simulink model "sschdlexZVSResonantConverterModel"  (R2026a)
settings: Solver=FixedStepDiscrete  StopTime=0.0001
libraries: fl_lib x9, nesl_utility x8, ee_lib x2
settings Model: DataTypeOverride=Off  Creator=The MathWorks, Inc.  LastModifiedBy=The MathWorks, Inc.
settings OptimizationCC: ConditionallyExecuteInputs=off
settings DebuggingCC: AlgebraicLoopMsg=error  SingleTaskRateTransMsg=error
settings HardwareCC: ProdHWDeviceType=ASIC/FPGA->ASIC/FPGA  TargetBitPerLong=64.0  TargetBitPerPointer=64.0  TargetBitPerSizeT=64.0  TargetBitPerPtrDiffT=64.0  TargetLongLongMode=on  TargetIntDivRoundTo=Zero  TargetEndianess=LittleEndian  TargetWordSize=64.0  TargetHWDeviceType=Custom Processor->MATLAB Host Computer  ProdEqTarget=off
settings SimscapeCC: SimscapeNominalValues="[{\"value\":\"1\",\"unit\":\"A\"},{\"value\":\"1\",\"unit\":\"bar\"},{\"value\":\"1\",\"unit\":\"cm^2\"},{\"value\":\"1\",\"unit\":\"cm^3/s\"},{\"value\":\"1\",\"unit\":\"kJ/kg\"},{\"value\":\"1\",\"unit\":\"kW\"},{\"value\":\"1\",\"unit\":\"l\"},{\"value\":\"1\",\"unit\":\"N\"},{\"value\":\"1\",\"unit\":\"N*m\"},{\"value\":\"1\",\"unit\":\"V\"}]"  SimscapeLogType=none  SimscapeLogDataHistory=5000.0

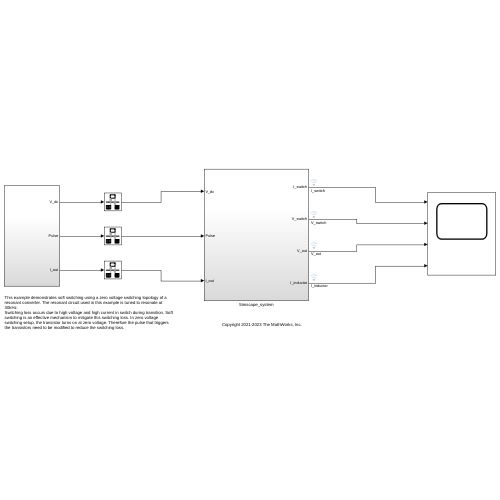
[thumbnail: Simulink's stored preview of the top-level diagram]
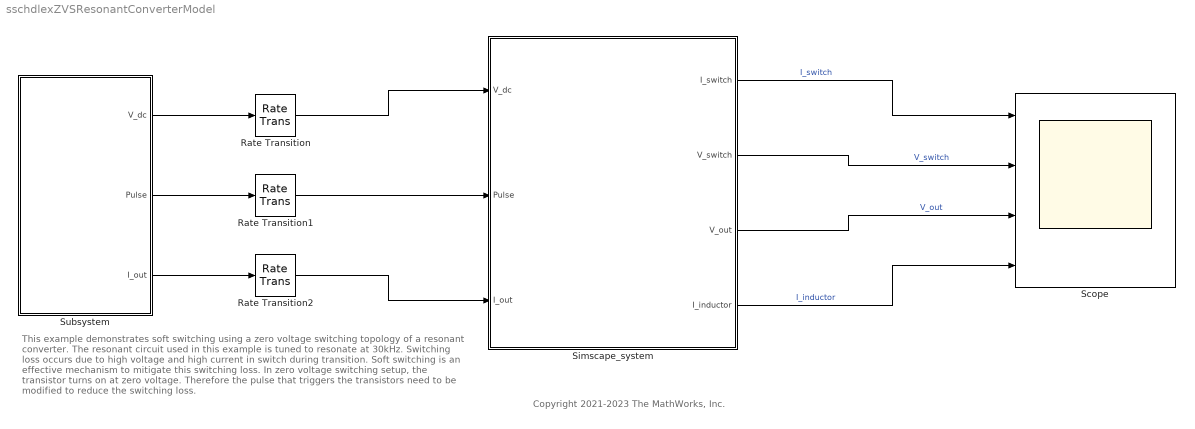
== system sschdlexZVSResonantConverterModel ==
  note: This example demonstrates soft switching using a zero voltage switching topology of a resonant converter. The resonant circuit used in this example is tuned to resonate at 30kHz.
      | Switching loss occurs due to high voltage and high current in switch during transition. Soft switching is an effective mechanism to mitigate this switching loss. In zero voltage switching setup, the transistor turns on at zero voltage. Therefore the pulse that triggers the transistors need to be modified to reduce the switching loss.
  note: Copyright 2021-2023 The MathWorks, Inc.
  Rate Transition : RateTransition
  Rate Transition1 : RateTransition
  Rate Transition2 : RateTransition
  Scope : Scope  NumInputPorts=4
      settings: ActiveDisplayYMinimum=-0.125  ActiveDisplayYMaximum=1.125
  Simscape_system : Subsystem
  Subsystem : Subsystem
  wires:
  Subsystem/1(V_dc) -> Rate Transition/1
  Subsystem/2(Pulse) -> Rate Transition1/1
  Subsystem/3(I_out) -> Rate Transition2/1
  Rate Transition/1 -> Simscape_system/1(V_dc)
  Rate Transition1/1 -> Simscape_system/2(Pulse)
  Rate Transition2/1 -> Simscape_system/3(I_out)
  Simscape_system/1(I_switch) -> Scope/1  "I_switch"
  Simscape_system/2(V_switch) -> Scope/2  "V_switch"
  Simscape_system/3(V_out) -> Scope/3  "V_out"
  Simscape_system/4(I_inductor) -> Scope/4  "I_inductor"

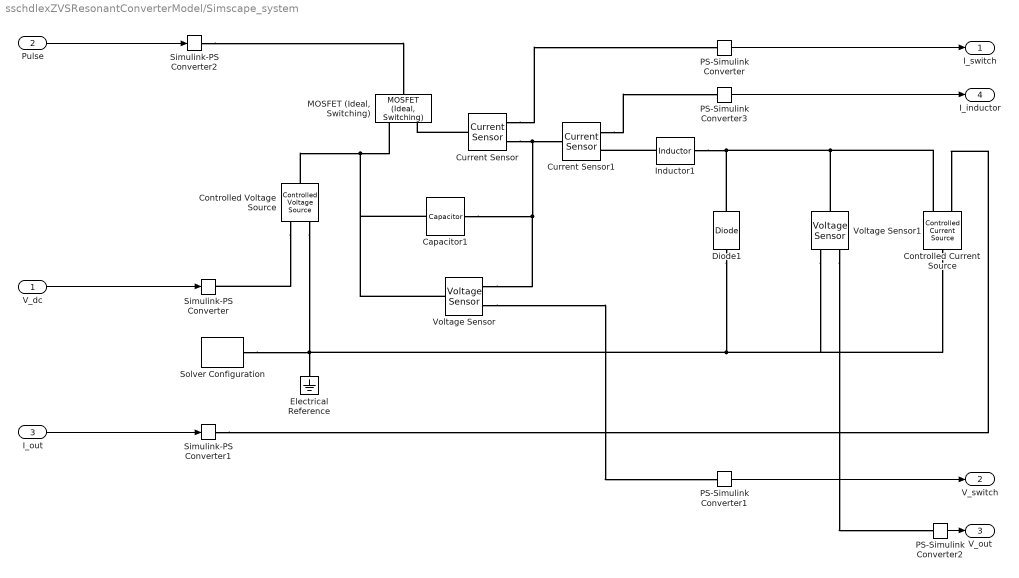
== system sschdlexZVSResonantConverterModel/Simscape_system ==
  V_dc : Inport
  Pulse : Inport  Port=2
  I_out : Inport  Port=3
  Capacitor1 : fl_lib/Electrical/Electrical Elements/Capacitor  c=0.1e-6 F  r=1e-6 Ohm  g=0 1/Ohm  i_specify=off  i_priority=None  i=0 A  i_nominal_specify=off  i_nominal_value=1  i_nominal_unit=A  v_specify=off  v_priority=None  v=0 V  v_nominal_specify=off  v_nominal_value=1  v_nominal_unit=V  vc_specify=off  vc_priority=High  vc=0 V  vc_nominal_specify=off  vc_nominal_value=1  vc_nominal_unit=V
  Controlled Current Source : fl_lib/Electrical/Electrical Sources/Controlled Current Source
  Controlled Voltage Source : fl_lib/Electrical/Electrical Sources/Controlled Voltage Source
  Current Sensor : fl_lib/Electrical/Electrical Sensors/Current Sensor
  Current Sensor1 : fl_lib/Electrical/Electrical Sensors/Current Sensor
  Diode1 : ee_lib/Semiconductors & Converters/Diode  ModelType=ee.enum.diode.modelType.pwl  TableType=ee.enum.diode.tableType.IfMat  IfMat=[.07, .12, .19, 1.75, 4.24, 7.32, 11.2; .16, .3, .72, 2.14, 5.02, 8.35, 13.12] A  VfMat=[.9, 1.15, 1.25, 1.5, 1.75, 2.17, 2.6, 2.85; .58, .68, .75, 1.1, 1.38, 1.77, 2.27, 2.7] V  TjVec=[25, 125] degC  VfVec=[.5, .7, .9, 1.3, 1.7, 2.1, 2.5] V  IfVec=[.1, .2, .5, 1, 2, 4, 7, 10] A  IrMat=[1e-06, 2e-06, 5e-06, 1e-05, 2.5e-05, 5e-05, .0001; 2e-06, 5e-06, 1e-05, 4e-05, 8e-05, .0002, .0005] A  VrMat=[10, 100, 200, 250, 300, 325, 350; 10, 70, 160, 220, 270, 300, 320] V  VrVec=[10, 20, 40, 50, 70, 80, 100] V  IrVec=[1e-06, 2e-06, 5e-06, 1e-05, 2e-05, 5e-05, .0001] A  Vf=0.6 V  Ron=0.3 Ohm  Goff=1e-8 S  prmExp=ee.enum.diode.expParam.useTwo  I12=[.0137, .545] A  V12=[.6, .7] V  RS=0 Ohm  Tmeas=25 degC  IS=1e-12 A  ec=1  I1=0.0137 A  V1=0.6 V  N_series=1  N_parallel=1  ZenerEnable=false  Rz=0.3 Ohm  BV=inf V  C_param=ee.enum.diode.capParam.fixed  CJ=0 pF  CJ0=5 pF  Vvec=[.1, 10, 100] V  Cvec=[3.5, 1, .4] pF  VJ=1 V  Mgrad=0.5  FC=0.5  Q_param=ee.enum.diode.recoveryParam.off  iRM=-7.15 A  iF=4 A  didt=-750 A/us  trr_factor=3  trr=115 ns  Qrr=150 nA*s  Vr=-600 V  Ls=150 nH  Erec=0.03 J  TT=50 ns  tau=100 ns  T_param=ee.enum.diode.temperatureParam.off  Tdevice=25 degC  I1_T2=0.245 A  V1_T2=0.5 V  IS_T2=1.25e-7 A  Tmeas2=125 degC  XTI_param=ee.enum.diode.xtiParam.pn  XTI=3  EG_param=ee.enum.diode.egapParam.material_si  EG=1.11 eV  dBVdT=0 V/K  enable_fault_input=simscape.enum.onoff.off  i_specify=off  i_priority=None  i=0 A  i_nominal_specify=off  i_nominal_value=1  i_nominal_unit=A  v_specify=off  v_priority=None  v=0 V  v_nominal_specify=off  v_nominal_value=1  v_nominal_unit=V  v_capacitor_specify=off  v_capacitor_priority=None  v_capacitor=0 V  v_capacitor_nominal_specify=off  v_capacitor_nominal_value=1  v_capacitor_nominal_unit=V  Qj_specify=off  Qj_priority=High  Qj=0 C  Qj_nominal_specify=off  Qj_nominal_value=1  Qj_nominal_unit=C  i_diode_specify=off  i_diode_priority=None  i_diode=0 A  i_diode_nominal_specify=off  i_diode_nominal_value=1  i_diode_nominal_unit=A  v_diode_specify=off  v_diode_priority=None  v_diode=0 V  v_diode_nominal_specify=off  v_diode_nominal_value=1  v_diode_nominal_unit=V  i_capacitor_specify=off  i_capacitor_priority=None  i_capacitor=0 A  i_capacitor_nominal_specify=off  i_capacitor_nominal_value=1  i_capacitor_nominal_unit=A  fidelity_level=ee.enum.diode.fidelity.includeChargeDyn  rec_loss_model=ee.enum.diode.reverseRecoveryModel.fixed  ErecVal=0 J  scaleWithIandV=true  ErecMat=zeros(2, 3) J  ErecMat3D=zeros(2, 3, 2) J  TjrecVec=[298.15, 398.15] K  IfrecVec=[.1, 1, 10] A  IrecVal=10 A  VrecVal=10 V  VrecVec=[0, 100] V  tFilter=1 / 1000 / 100 s  thermal_network_parameterization=ee.enum.thermalNetworkTopology.junctionCase  Rth=[0, 10] K/W  Rth_Cauer=[1, 3, 10] K/W  Rth_Foster=[4, 6] K/W  thermal_mass_parameterization=ee.enum.thermalNetwork.timeconstant  thermal_mass=[0, 1] J/K  thermal_mass_Cauer=[.1, .3, 1] J/K  thermal_mass_Foster=[1.5, 3] J/K  thermal_time_constant=[0, 10] s  thermal_time_constant_Cauer=[1, 3, 10] s  thermal_time_constant_Foster=[6, 18] s  thermal_mass_initial_temperatures=[25, 25] degC  thermal_mass_initial_temperatures_Cauer=[25, 25, 25] degC  junction_thermal_mass=0.01 J/K  Tvec_initial_Foster=[25, 25, 25, 25] degC  no_thermal_network=0  junction_temperature_specify=off  junction_temperature_priority=None  junction_temperature=25 degC  junction_temperature_nominal_specify=off  junction_temperature_nominal_value=1  junction_temperature_nominal_unit=degC
  Electrical Reference : fl_lib/Electrical/Electrical Elements/Electrical Reference
  Inductor1 : fl_lib/Electrical/Electrical Elements/Inductor  l=0.1e-3 H  r=0 Ohm  g=1e-9 1/Ohm  i_specify=on  i_priority=None  i=1 A  i_nominal_specify=off  i_nominal_value=1  i_nominal_unit=A  v_specify=off  v_priority=None  v=0 V  v_nominal_specify=off  v_nominal_value=1  v_nominal_unit=V  i_L_specify=off  i_L_priority=High  i_L=0 A  i_L_nominal_specify=off  i_L_nominal_value=1  i_L_nominal_unit=A
  "MOSFET (Ideal, Switching)" : ee_lib/Semiconductors & Converters/MOSFET (Ideal, Switching)  port_option=ee.enum.controlport.ps  Rds=1 Ohm  Goff=1e-6 1/Ohm  Vth=0.7 V  diode_param=2  diode_Vf=0.8 V  diode_Ron=0.001 Ohm  diode_Goff=1e-5 1/Ohm  diode_C=50e-9 F  diode_iRM=-235 A  diode_iF=300 A  diode_idot=-50 A/us  diode_trr_param=1  diode_trr_factor=3  diode_trr=15 us  diode_Qrr=1500 s*uA  ids_specify=off  ids_priority=None  ids=0 A  ids_nominal_specify=off  ids_nominal_value=1  ids_nominal_unit=A  vds_specify=off  vds_priority=None  vds=0 V  vds_nominal_specify=off  vds_nominal_value=1  vds_nominal_unit=V  vgs_specify=off  vgs_priority=None  vgs=0 V  vgs_nominal_specify=off  vgs_nominal_value=1  vgs_nominal_unit=V  thermal_loss_option=ee.enum.converters.thermalLossOption.constantvalues  Von_data=[0, 1.8, 3.2, 6, 10, 16; 0, 2, 5.5, 9.5, 15, 25] V  Tj=[298.15, 448.15] K  Iout_data=[0, 20, 40, 60, 80, 100] A  tabulateWithVds=false  Eon_data=[0, 55.04, 124.57, 235.53, 362.12; 0, 71.25, 161.25, 304.88, 468.75] * 1e-6 J  Eoff_data=[0, 18, 30, 56.1, 76.5; 0, 22.5, 37.5, 70.13, 95.63] * 1e-6 J  Eon_data_3D=[zeros(2, 5, 3)] J  Eoff_data_3D=[zeros(2, 5, 3)] J  Tj_loss=[298.15, 448.15] K  Iout_data_loss=[0, 10, 20, 30, 40] A  Vds_loss=[0, 150, 300] V  Eon_scalar=22.86e-3 J  Eoff_scalar=17.14e-3 J  Voff=300 V  Iout_scalar=600 A  useCurrentFromPreviousCycle=false  useVoltageFromPreviousCycle=false  diodeModelType=ee.enum.converters.diodeModelType.pwl  diodeTableType=ee.enum.diode.tableType.IfMat  diode_ReverseIVType=ee.enum.diode.diodeReverseIV.constant  diode_IfMat=[.07, .12, .19, 1.75, 4.24, 7.32, 11.2; .16, .3, .72, 2.14, 4.02, 6.35, 9.12] A  diode_VfMat=[.9, 1.15, 1.25, 1.5, 1.75, 2.17, 2.6, 2.85; .58, .68, .75, 1.1, 1.38, 1.77, 2.27, 2.7] V  diode_TjVec=[25, 125] degC  diode_VfVec=[.5, .7, .9, 1.3, 1.7, 2.1, 2.5] V  diode_IfVec=[.1, .2, .5, 1, 2, 4, 7, 10] A  diode_IrMat=[1e-06, 2e-06, 5e-06, 1e-05, 2.5e-05, 5e-05, .0001; 2e-06, 5e-06, 1e-05, 4e-05, 8e-05, .0002, .0005] A  diode_VrMat=[10, 100, 200, 250, 300, 325, 350; 10, 70, 160, 220, 270, 300, 320] V  diode_VrVec=[10, 20, 40, 50, 70, 80, 100] V  diode_IrVec=[1e-06, 2e-06, 5e-06, 1e-05, 2e-05, 5e-05, .0001] A  diode_Vr=-600 V  diode_Ls=150 nH  diode_Erec=0.03 J  diode_rec_loss_model=ee.enum.diode.reverseRecoveryModel.fixed  diode_ErecVal=0 J  diode_scaleWithIandV=true  diode_ErecMat=zeros(2, 3) J  diodeErecMat3D=zeros(2, 3, 2) J  diode_TjrecVec=[298.15, 398.15] K  diode_IfrecVec=[.1, 1, 10] A  diodeVrecVec=[0, 100] V  diode_IrecVal=10 A  diode_VrecVal=10 V  diode_tFilter=1 / 1000 / 100 s  separateThermalPortForDiode=false  thermal_network_parameterization=ee.enum.thermalNetworkTopology.external  Rth=[.03, .2] K/W  Rth_Cauer=[.03, .1, .2] K/W  Rth_Foster=[.03, .2] K/W  thermal_mass_parameterization=ee.enum.thermalNetwork.timeconstant  thermal_mass=[3, 25] J/K  thermal_mass_Cauer=[3, 10, 25] J/K  thermal_mass_Foster=[33, 50] J/K  thermal_time_constant=[.1, 5] s  thermal_time_constant_Cauer=[.1, 1, 5] s  thermal_time_constant_Foster=[1, 10] s  thermal_mass_initial_temperatures=[25, 25] degC  thermal_mass_initial_temperatures_Cauer=[25, 25, 25] degC  junction_thermal_mass=0.1 J/K  Tvec_initial_Foster=[25, 25, 25, 25] degC  RthDiode=[.03, .2] K/W  RthCauerDiode=[.03, .1, .2] K/W  RthFosterDiode=[.03, .2] K/W  thermalMassDiode=[3, 25] J/K  thermalMassCauerDiode=[3, 10, 25] J/K  thermalMassFosterDiode=[33, 50] J/K  thermalTauDiode=[.1, 5] s  thermalTauCauerDiode=[.1, 1, 5] s  thermalTauFosterDiode=[1, 10] s  thermalMassInitTempDiode=[25, 25] degC  thermalMassInitTempCauerDiode=[25, 25, 25] degC  junctionthermalMassDiode=0.1 J/K  TVecInitialFosterDiode=[25, 25, 25, 25] degC  no_thermal_network=0  mosfet_junction_temperature_specify=off  mosfet_junction_temperature_priority=None  mosfet_junction_temperature=25 degC  mosfet_junction_temperature_nominal_specify=off  mosfet_junction_temperature_nominal_value=1  mosfet_junction_temperature_nominal_unit=degC  diode_junction_temperature_specify=off  diode_junction_temperature_priority=None  diode_junction_temperature=25 degC  diode_junction_temperature_nominal_specify=off  diode_junction_temperature_nominal_value=1  diode_junction_temperature_nominal_unit=degC  Qj_specify=off  Qj_priority=None  Qj=0 W  Qj_nominal_specify=off  Qj_nominal_value=1  Qj_nominal_unit=W  accumulatedSwitchingLosses_specify=off  accumulatedSwitchingLosses_priority=None  accumulatedSwitchingLosses=0 J
  PS-Simulink Converter{,1..3} (4 alike) : nesl_utility/PS-Simulink Converter  PhysicalDomain=network_engine_domain  SubClassName=ps_output  LeftPortType=input  RightPortType=output  PseudoPeriodic=off  Frequencies=[]  VectorFormat=1-D array  Unit=inherit  AffineConversion=off
  Simulink-PS Converter : nesl_utility/Simulink-PS Converter  PhysicalDomain=network_engine_domain  SubClassName=ps_input  LeftPortType=input  RightPortType=output  PseudoPeriodic=off  Frequencies=[]  NoiseDistribution=none  NoiseParameters=[]  Unit=1  AffineConversion=off  FilteringAndDerivatives=provide  SimscapeFilterOrder=1  InputFilterTimeConstant=0.001  UdotUserProvided=0
  Simulink-PS Converter1 : nesl_utility/Simulink-PS Converter  PhysicalDomain=network_engine_domain  SubClassName=ps_input  LeftPortType=input  RightPortType=output  PseudoPeriodic=off  Frequencies=[]  NoiseDistribution=none  NoiseParameters=[]  Unit=1  AffineConversion=off  FilteringAndDerivatives=provide  SimscapeFilterOrder=1  InputFilterTimeConstant=0.001  UdotUserProvided=0
  Simulink-PS Converter2 : nesl_utility/Simulink-PS Converter  PhysicalDomain=network_engine_domain  SubClassName=ps_input  LeftPortType=input  RightPortType=output  PseudoPeriodic=off  Frequencies=[]  NoiseDistribution=none  NoiseParameters=[]  Unit=1  AffineConversion=off  FilteringAndDerivatives=provide  SimscapeFilterOrder=1  InputFilterTimeConstant=0.001  UdotUserProvided=0
  Solver Configuration : nesl_utility/Solver Configuration  PhysicalDomain=network_engine_domain  SubClassName=solver  LeftPortType=input  RightPortType=generic  Tones=[]  Harmonics=[]  SimulateNoise=off  Profile=off  UseLocalSampling=off  EnableSwitchedLinearOptims=on  FrequencyDomain=off  UseCCode=off  RelTol=0.001  AbsTol=1e-06  MinStep=1e-09  ToWorkspace=off  RevertToSquareIcSolve=off  NumHomotopyIterations=100  PhasorMode=off  PhasorModeNumHarmonics=1  ConsistencySolver=NEWTON_FTOL  CanonicalOrdering=UNORDERED  OptimizeIntermediates=UNOPTIMIZED  IndexReductionMethod=DerivativeReplacement  DoDC=off  ResidualTolerance=1e-09  ConsistencyTolSource=GLOBAL  ConsistencyAbsTol=0.001  ConsistencyRelTol=0.001  ConsistencyTolFactor=0.001  UseLocalSolver=on  LocalSolverChoice=NE_BACKWARD_EULER_ADVANCER  ResolveIndetEquations=on  FunctionEvalNumThread=1  LocalSolverSampleTime=1e-6  DoFixedCost=on  MaxNonlinIter=2  MaxModeIter=2  ComputeImpulses=off  ImpulseIterations=1  LinearAlgebra=auto  LinearAlgebraNumThread=0  EquationFormulation=NE_TIME_EF  DelaysMemoryBudget=1024  AutomaticFiltering=on  FilteringTimeConstant=0.001  PartitionStorageMethod=AS_NEEDED  PartitionMemoryBudget=1024  PartitionMethod=ROBUST  MultibodyUseLocalSolver=off  MultibodyLocalSolverChoice=ODE1  MultibodyLocalSolverSampleTime=0.001
  Voltage Sensor : fl_lib/Electrical/Electrical Sensors/Voltage Sensor
  Voltage Sensor1 : fl_lib/Electrical/Electrical Sensors/Voltage Sensor
  I_switch : Outport
  V_switch : Outport  Port=2
  V_out : Outport  Port=3
  I_inductor : Outport  Port=4
  wires:
  I_out/1 -> Simulink-PS Converter1/1
  PS-Simulink Converter1/1 -> V_switch/1
  Pulse/1 -> Simulink-PS Converter2/1
  PS-Simulink Converter2/1 -> V_out/1
  PS-Simulink Converter/1 -> I_switch/1
  V_dc/1 -> Simulink-PS Converter/1
  PS-Simulink Converter3/1 -> I_inductor/1
  connections:
  Current Sensor/RConn1 -- PS-Simulink Converter/LConn1
  Current Sensor/LConn1 -- "MOSFET (Ideal, Switching)"/RConn2
  Current Sensor/RConn2 -- Voltage Sensor/RConn2 -- Capacitor1/RConn1 -- Current Sensor1/LConn1
  Controlled Voltage Source/RConn2 -- Diode1/LConn1 -- Voltage Sensor1/RConn2 -- Controlled Current Source/LConn1 -- Electrical Reference/LConn1 -- Solver Configuration/RConn1
  Voltage Sensor1/RConn1 -- PS-Simulink Converter2/LConn1
  Controlled Current Source/RConn2 -- Diode1/RConn1 -- Inductor1/RConn1 -- Voltage Sensor1/LConn1
  Simulink-PS Converter1/RConn1 -- Controlled Current Source/RConn1
  Controlled Voltage Source/RConn1 -- Simulink-PS Converter/RConn1
  Controlled Voltage Source/LConn1 -- Voltage Sensor/LConn1 -- Capacitor1/LConn1 -- "MOSFET (Ideal, Switching)"/RConn1
  Voltage Sensor/RConn1 -- PS-Simulink Converter1/LConn1
  Simulink-PS Converter2/RConn1 -- "MOSFET (Ideal, Switching)"/LConn1
  Inductor1/LConn1 -- Current Sensor1/RConn2
  Current Sensor1/RConn1 -- PS-Simulink Converter3/LConn1

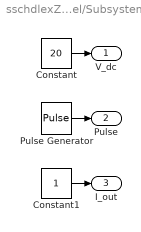
== system sschdlexZVSResonantConverterModel/Subsystem ==
  Constant : Constant  Value=20  SampleTime=0
  Constant1 : Constant  SampleTime=0
  Pulse Generator : DiscretePulseGenerator  Period=30  PulseWidth=16  SampleTime=1e-6
  V_dc : Outport
  Pulse : Outport  Port=2
  I_out : Outport  Port=3
  wires:
  Pulse Generator/1 -> Pulse/1
  Constant/1 -> V_dc/1
  Constant1/1 -> I_out/1
